simulink subsystem "uart"  (R2023a)
settings: Solver=VariableStepAuto  StartTime=0.0  StopTime=10.0  RelTol=1e-3
undefined symbols (not defined in the file or in its folder): LF
libraries: instrumentseriallib x3
settings Model: Creator=Westar  LastModifiedBy=Westar
settings RTWCC: GPUComputeCapability=5.0

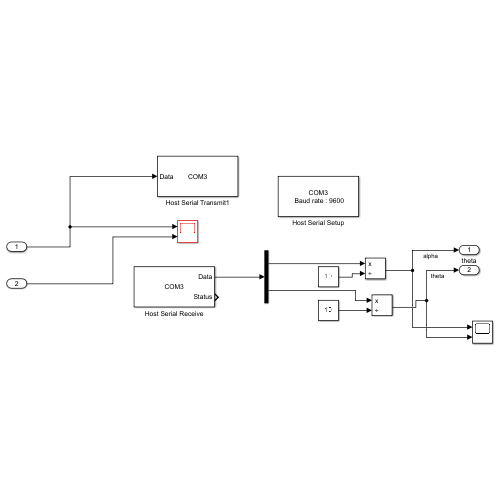
[thumbnail: Simulink's stored preview of the top-level diagram]
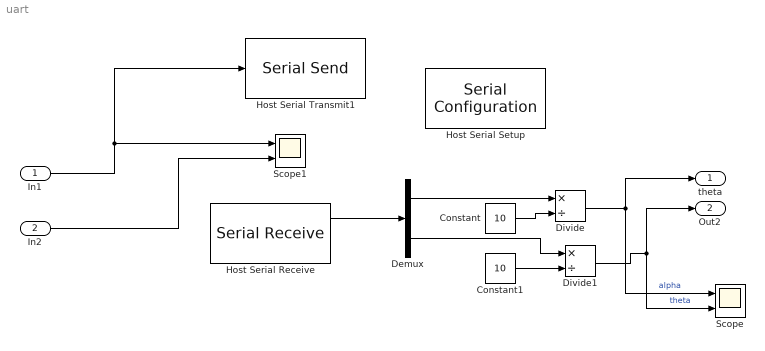
== system uart ==
  In1 : Inport
  In2 : Inport  Port=2
  Constant : Constant  Value=10
  Constant1 : Constant  Value=10
  Demux : Demux  Outputs=2
  Divide : Product  Inputs=*/  OutDataTypeStr=single
  Divide1 : Product  Inputs=*/  OutDataTypeStr=single
  Host Serial Receive : instrumentseriallib/Serial Receive  PortSel=COM3  Port=COM3  ComPort=COM3  DataType=int8  SaveDataType=uint8  ToggleHeader=on  Header='A'  ToggleTerminator=on  Terminator=LF ('\n')  CustomTerminator='E'  InputFormat=Row major  ToggleDataSize=on  DataSize=2  EnableBlockingMode=off  ActionDataUnavailable=Output last received value  ActionWhenDataUnavailable=Output last received value  CustomValue=0  SampleTime=-1  SimulateUsing=Interpreted execution  BlockInModel=on  aMode=5
      settings: LibrarySourceBlock=mcblib/Protection and Diagnostics/Host Serial Receive
  Host Serial Setup : instrumentseriallib/Serial Configuration  Priority=-99  PortSel=COM3  Port=COM3  ComPort=COM3  BaudRate=9600  DataBits=8  Parity=none  StopBits=1  ByteOrder=little-endian  FlowControl=none  Timeout=1.0  SimulateUsing=Interpreted execution  BlockInModel=on  aMode=5
      settings: LibrarySourceBlock=mcblib/Protection and Diagnostics/Host Serial Setup
  Host Serial Transmit1 : instrumentseriallib/Serial Send  PortSel=COM3  Port=COM3  ComPort=COM3  Header='S'  Terminator=Custom terminator  CustomTerminator='E'  EnableBlockingMode=off  SimulateUsing=Interpreted execution  BlockInModel=on  aMode=5
      settings: LibrarySourceBlock=mcblib/Protection and Diagnostics/Host Serial Transmit
  Scope : Scope  NumInputPorts=2
  Scope1 : Scope  NumInputPorts=2
  theta : Outport  OutDataTypeStr=single
  Out2 : Outport  Port=2  OutDataTypeStr=single
  wires:
  Demux/2 -> Divide1/1
  Host Serial Receive/1 -> Demux/1
  Constant1/1 -> Divide1/2
  Demux/1 -> Divide/1
  Divide1/1 -> Out2/1, Scope/2  "theta"
  Constant/1 -> Divide/2
  Divide/1 -> theta/1, Scope/1  "alpha"
  In2/1 -> Scope1/2
  In1/1 -> Scope1/1, Host Serial Transmit1/1
